simulink model "mcb_pmsm_foc_qep_f28379d_SIUnit"  (R2025b)
settings: Solver=FixedStepDiscrete  StartTime=0.0  StopTime=4  RelTol=1e-3  EnableMultiTasking=on
InitFcn:
  | mcb_pmsm_foc_qep_f28379d_SIUnit_data;
values from neighbouring files (symbols this model uses):
  A = [ -Rs/L,           0,                  0 ... (first row only)    [mcb_pmsm_fsfb_f28379d_param.m]    (also in v0_pmsm_fsfb_sim_for_flipsky_.m = [; v1_0_3_sim_param_fsfc.m = [)
  dataType = 'single'    [mcb_pmsm_foc_qep_f28379d_SIUnit_data.m]
  inverter = mcb.updateInverterParameters(pmsm,inverter,target)    [mcb_pmsm_foc_qep_f28379d_SIUnit_data.m]
  lambda_pm = pmsm.FluxPM    [mcb_pmsm_foc_qep_f28379d_SIUnit_data.m]
  PI_params = mcb.calcFOCGains(motor,Ts,Ts_speed,SpdLPFltCoeff=LPFltCoeff)    [mcb_pmsm_foc_qep_f28379d_SIUnit_data.m]
  pmsm = mcb.getPMSMParameters('Teknic2310P')    [mcb_pmsm_foc_qep_f28379d_SIUnit_data.m]
  T_pwm = 1/PWM_frequency    (= 5e-05)    [mcb_pmsm_foc_qep_f28379d_SIUnit_data.m]
  target = mcb.getProcessorParameters('F28379D',PWM_frequency)    [mcb_pmsm_foc_qep_f28379d_SIUnit_data.m]
  Ts = T_pwm    (= 5e-05)    [mcb_pmsm_foc_qep_f28379d_SIUnit_data.m]    (also in v0_pmsm_fsfb_sim_for_flipsky_.m = 0.0001; v1_0_3_sim_param_fsfc.m = 0.0001)
  Ts_inverter = T_pwm/2    (= 2.5e-05)    [mcb_pmsm_foc_qep_f28379d_SIUnit_data.m]
  Ts_motor = T_pwm/2    (= 2.5e-05)    [mcb_pmsm_foc_qep_f28379d_SIUnit_data.m]
  Ts_simulink = T_pwm/2    (= 2.5e-05)    [mcb_pmsm_foc_qep_f28379d_SIUnit_data.m]
  Ts_speed = 10*Ts    (= 0.0005)    [mcb_pmsm_foc_qep_f28379d_SIUnit_data.m]
undefined symbols (not defined in the file or in its folder): bit, DiscIntNeverNeededParam, Down, GPTRIP1SEL, GPTRIP2SEL, TZ1, TZ2, Up
libraries: mcbcontrolslib x8, c2802xlib x7, simulink x7, c280xlib x5, c2837xDlib x4, mcbeeMathTransformLib x3, slpidlib x3, mcbpositiondecoderlib x3, c2000lib x1, svdutilitieslib x1, autolibpmsmexterior x1
(part 2 of 2)

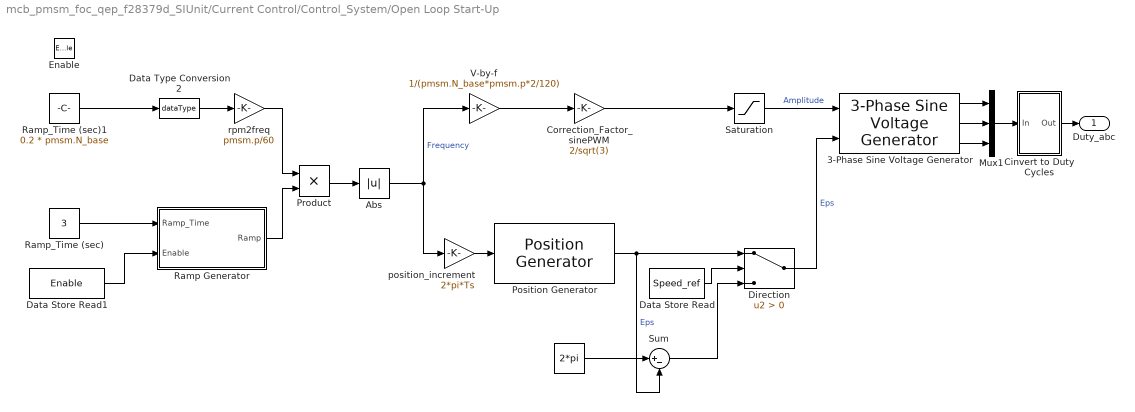
== system mcb_pmsm_foc_qep_f28379d_SIUnit/Current Control/Control_System/Open Loop Start-Up ==
  Enable : EnablePort  StatesWhenEnabling=reset
  " " : Constant  Value=2*pi  OutDataTypeStr=dataType  SampleTime=-1
  3-Phase Sine Voltage Generator : mcbcontrolslib/3-Phase Sine Voltage Generator  AngleInput=Radians  N_points=1024
  Abs : Abs  SaturateOnIntegerOverflow=off
  Cinvert to Duty Cycles : Subsystem
  Correction_Factor_sinePWM : Gain  Gain=2/sqrt(3)  RndMeth=Simplest  OutDataTypeStr=Inherit: Same as input
  Data Store Read : DataStoreRead  DataStoreName=Speed_ref  IndexOptions=Index vector (dialog)  Indices=1  OutputSizes=1
  Data Store Read1 : DataStoreRead  DataStoreName=Enable  IndexOptions=Index vector (dialog)  Indices=1  OutputSizes=1
  Data Type Conversion2 : DataTypeConversion  OutDataTypeStr=dataType  RndMeth=Simplest  SaturateOnIntegerOverflow=off
  Direction : Switch  Criteria=u2 > Threshold  OutDataTypeStr=dataType  RndMeth=Simplest  SaturateOnIntegerOverflow=off  InputSameDT=off
  Mux1 : Mux  Inputs=3
  Position Generator : mcbcontrolslib/Position Generator  AngleOutput=Radians  InitialThetaSource=Specify via dialog  ExternalReset=none  Offset=0
  Product : Product  RndMeth=Simplest  OutDataTypeStr=Inherit: Same as first input
  Ramp Generator : Subsystem
  Ramp_Time (sec) : Constant  Value=3  OutDataTypeStr=dataType  SampleTime=-1
  Ramp_Time (sec)1 : Constant  Value=0.2 * pmsm.N_base  OutDataTypeStr=dataType  SampleTime=-1
  Saturation : Saturate  UpperLimit=0.95  LowerLimit=0.15  RndMeth=Simplest
  Sum : Sum  Inputs=|+-  RndMeth=Simplest  OutDataTypeStr=Inherit: Same as first input
  V-by-f : Gain  Gain=1/(pmsm.N_base*pmsm.p*2/120)  RndMeth=Simplest  OutDataTypeStr=Inherit: Same as input
  position_increment : Gain  Gain=2*pi*Ts  RndMeth=Simplest  OutDataTypeStr=Inherit: Same as input
  rpm2freq : Gain  Gain=pmsm.p/60  RndMeth=Simplest  OutDataTypeStr=Inherit: Same as input
  Duty_abc : Outport  VectorParamsAs1DForOutWhenUnconnected=off
  wires:
  3-Phase Sine Voltage Generator/1 -> Mux1/1
  3-Phase Sine Voltage Generator/3 -> Mux1/3
  Direction/1 -> 3-Phase Sine Voltage Generator/2  "Eps"
  Saturation/1 -> 3-Phase Sine Voltage Generator/1  "Amplitude"
  Ramp Generator/1(Ramp) -> Product/2
  Ramp_Time (sec)/1 -> Ramp Generator/1(Ramp_Time)
  Position Generator/1 -> Sum/2, Direction/1  "Eps"
  " "/1 -> Sum/1
  Sum/1 -> Direction/3
  Abs/1 -> position_increment/1, V-by-f/1  "Frequency"
  position_increment/1 -> Position Generator/1
  V-by-f/1 -> Correction_Factor_sinePWM/1
  Product/1 -> Abs/1
  rpm2freq/1 -> Product/1
  Data Store Read1/1 -> Ramp Generator/2(Enable)
  Correction_Factor_sinePWM/1 -> Saturation/1
  3-Phase Sine Voltage Generator/2 -> Mux1/2
  Data Type Conversion2/1 -> rpm2freq/1
  Ramp_Time (sec)1/1 -> Data Type Conversion2/1
  Data Store Read/1 -> Direction/2
  Mux1/1 -> Cinvert to Duty Cycles/1(In)
  Cinvert to Duty Cycles/1(Out) -> Duty_abc/1

== system mcb_pmsm_foc_qep_f28379d_SIUnit/Current Control/HW_Inputs/Sensor Driver Blocks (codegen) ==
  Sim : Inport
  ADC_B_IN2 : c2802xlib/ADC  blkParamProc=C2000_Type4  ADCModule=B  samplingMode=Single sample mode  ADCResolution=12-bit (Single-ended input)  useSOC1=SOC0  useSOC2=SOC0_SOC1  SOCAcquisitionWindow=15  SOCTriggerSource=ePWM1_ADCSOCA  SOCInterruptTrigger=No ADCINT  Ts=-1  dType=uint16  postInterrupt=on  interruptSel=ADCINT1  ADCINTContinuous=on  endma=off  chdma=1  conv1=ADCINA0  conv2=ADCINA0 and ADCINB0  conv1_Type4=ADCIN2  conv2_Type4=ADCIN0 and ADCIN1
  ADC_C_IN2 : c2802xlib/ADC  blkParamProc=C2000_Type4  ADCModule=C  samplingMode=Single sample mode  ADCResolution=12-bit (Single-ended input)  useSOC1=SOC0  useSOC2=SOC0_SOC1  SOCAcquisitionWindow=15  SOCTriggerSource=ePWM1_ADCSOCA  SOCInterruptTrigger=No ADCINT  Ts=-1  dType=uint16  postInterrupt=off  interruptSel=ADCINT1  ADCINTContinuous=on  endma=off  chdma=1  conv1=ADCINA0  conv2=ADCINA0 and ADCINB0  conv1_Type4=ADCIN2  conv2_Type4=ADCIN0 and ADCIN1
  Mux1 : Mux
  Terminator : Terminator
  eQEP : c280xlib/eQEP  useModule=eQEP1  pcInputmode=Quadrature-count  externalClockrate=2x resolution: Count the rising/falling edge  swapPolarityselection=Clockwise  qdfOutputport=off  qapPolarityselection=on  qbpPolarityselection=on  qipPolarityselection=on  qspPolarityselection=off  igatePolarityselection=off  sampleTime=-1  pcOutputport=on  pcMaximumvalue=2^16-1  indexInitializationcheck=off  indexInitializationevent=Rising edge  strobeInitializationcheck=off  strobeInitializationevent=Rising edge  softwareInitializationcheck=off  softwareInitializationsource=Set to init value at start up  softwareInitializationmode=on  pcInitialvalue=2147483648  pcResetmode=Reset on the first index event  ieloutputport=on  indexEventlatch=Falling edge  seloutputport=off  strobeEventlatch=Rising edge  pcefOutputport=off  enableEqepcapture=off  qctmrOutputport=off  qcprdOutputport=off  captureTimerprescaler=128  upEventprescaler=128  overflowErrorflag=off  directionErrorflag=off  captureTimerposition=On position counter read  unitTimerperiod=100000000  captureTimerlatch=off  capturePeriodlatch=off  positionCounterlatch=off  soenPolarityselection=off  spselPolarityselection=Index pin is used for sync output  compareValuesource=Specify via dialog  shadowMode=Load on QPOSCNT=0  compareValue=4294967295  syncOutputwidth=1  polaritySyncoutput=Active high  watchdogEnable=off  watchdogTimer=65535  outport1Datatype=auto  outport2Datatype=auto  outport3Datatype=auto  outport4Datatype=auto  outport5Datatype=auto  outport6Datatype=auto  outport7Datatype=auto  outport8Datatype=auto  outport9Datatype=auto  outport10Datatype=auto  outport11Datatype=auto  outport12Datatype=auto  eqepinterrupt_pce=off  eqepinterrupt_qpe=off  eqepinterrupt_qdc=off  eqepinterrupt_wto=off  eqepinterrupt_pcu=off  eqepinterrupt_pco=off  eqepinterrupt_pcr=off  eqepinterrupt_pcm=off  eqepinterrupt_sel=off  eqepinterrupt_iel=off  eqepinterrupt_uto=off  pheOutputport=off  watchdogOutputport=off  outport13Datatype=auto  outport14Datatype=auto
  Out : Outport
  wires:
  ADC_C_IN2/1 -> Mux1/1
  Mux1/1 -> Out/1
  ADC_B_IN2/1 -> Mux1/2
  Sim/1 -> Terminator/1
  eQEP/1 -> Mux1/3
  eQEP/2 -> Mux1/4

== system mcb_pmsm_foc_qep_f28379d_SIUnit/Current Control/HW_Inputs/Sensor Driver Blocks (sim) ==
  Sim : Inport
  Out : Outport
  wires:
  Sim/1 -> Out/1

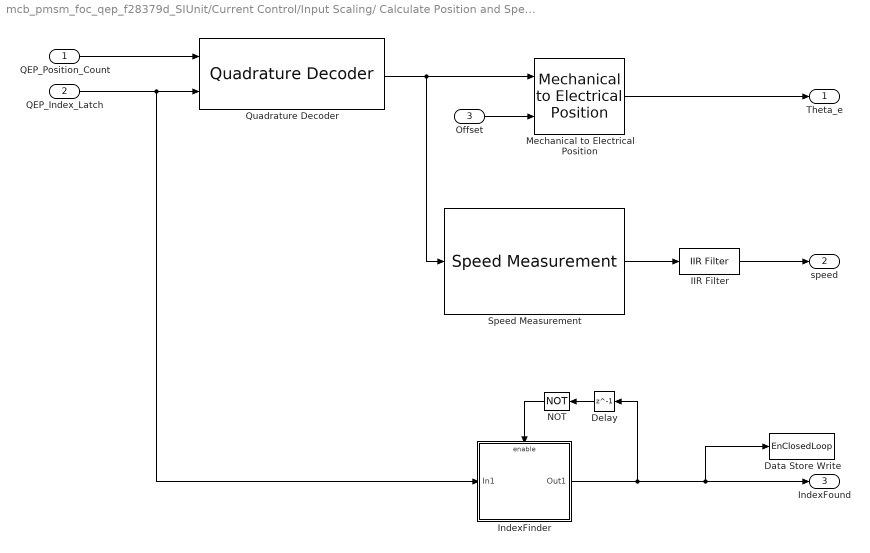
== system mcb_pmsm_foc_qep_f28379d_SIUnit/Current Control/Input Scaling/ Calculate Position and Speed ==
  QEP_Position_Count : Inport
  QEP_Index_Latch : Inport  Port=2
  Offset : Inport  Port=3
  Data Store Write : DataStoreWrite  DataStoreName=EnClosedLoop  IndexOptions=Index vector (dialog)  Indices=1  OutputSizes=1
  Delay : Delay  DelayLength=1
  IIR Filter : mcbcontrolslib/IIR Filter  VariantControl=Low Pass Filter  VariantSelect=Low-pass  FilterConstantInputType=Specify via dialog  Filter_constant=0.01  InitialOutput=Specify via dialog  InitialOutputValue=0  ExternalReset=none  advancedSettings=off  Ts=50e-6  cutOff_freq=32.1525
  IndexFinder : Subsystem
  Mechanical to Electrical Position : mcbpositiondecoderlib/Mechanical to Electrical Position  PolePairsInputType=Specify via dialog  NrPP=pmsm.p  selectedRange=Radians  MechOfstInputType=Input port  mechOffsetIn=0  maxAngleIn=2*pi  InputDataType=dataType  VariantSelect=floating-point
  NOT : Logic  Operator=NOT  AllPortsSameDT=off  OutDataTypeStr=boolean
  Quadrature Decoder : mcbpositiondecoderlib/Quadrature Decoder  ParameterInputType=off  CountsPerRevInverseDataType=single  EncoderSlitsPerRevolution=pmsm.QEPSlits  EncoderCountsPerSlit=4  CounterSize=16 bits  ExternalIndexCount=on  PositionUnit=Radians  PositionDataType=dataType
  Speed Measurement : mcbpositiondecoderlib/Speed Measurement  DiscreteStepInput=off  LastDiscreteStepInput=off  PositionUnit=Radians  PositionScalingDatatype=uint32  SpeedCalculationMode=Time interval for speed calculation  TempSpeedCalculationMode=Time interval for speed calculation  SampleTimeAsync=Ts  MaximumApplicationSpeed=6000  SpeedResolution=5e-6  DelayLength=20  MaximumMeasurableSpeed=29999  MeasurableSpeedResolution=1.397e-05  SpeedUnit=Radians/Sec  TempSpeedUnit=RPM  PerUnitSpeed=PU_System.N_base  SpeedDataType=dataType
  Theta_e : Outport  VectorParamsAs1DForOutWhenUnconnected=off
  speed : Outport  Port=2  VectorParamsAs1DForOutWhenUnconnected=off
  IndexFound : Outport  Port=3  InitialOutput=0  VectorParamsAs1DForOutWhenUnconnected=off
  wires:
  Speed Measurement/1 -> IIR Filter/1
  Mechanical to Electrical Position/1 -> Theta_e/1
  QEP_Position_Count/1 -> Quadrature Decoder/1
  Quadrature Decoder/1 -> Speed Measurement/1, Mechanical to Electrical Position/1
  Offset/1 -> Mechanical to Electrical Position/2
  IIR Filter/1 -> speed/1
  Delay/1 -> NOT/1
  NOT/1 -> IndexFinder/Enable
  IndexFinder/1(Out1) -> Data Store Write/1, IndexFound/1, Delay/1
  QEP_Index_Latch/1 -> IndexFinder/1(In1), Quadrature Decoder/2

== system mcb_pmsm_foc_qep_f28379d_SIUnit/Current Control/Input Scaling/Calculate Phase Currents ==
  Ia_ADC : Inport
  Ib_ADC : Inport  Port=2
  Add : Sum  Inputs=-+
  Data Store Read1 : DataStoreRead  DataStoreName=IaOffset  IndexOptions=Index vector (dialog)  Indices=1  OutputSizes=1
  Data Store Read2 : DataStoreRead  DataStoreName=IbOffset  IndexOptions=Index vector (dialog)  Indices=1  OutputSizes=1
  Data Type Conversion : DataTypeConversion  OutDataTypeStr=int32  ConvertRealWorld=Stored Integer (SI)  RndMeth=Simplest  SaturateOnIntegerOverflow=off
  Get ADC Voltage : Gain  Gain=target.ADC_Vref /target.ADC_MaxCount  OutDataTypeStr=dataType  RndMeth=Simplest
  Get Currents : Gain  Gain=inverter.invertingAmp/inverter.ISenseVoltPerAmp  RndMeth=Simplest  OutDataTypeStr=Inherit: Same as input
  Mux : Mux  Inputs=2
  Mux1 : Mux  Inputs=2
  Iab_meas : Outport  VectorParamsAs1DForOutWhenUnconnected=off
  wires:
  Data Type Conversion/1 -> Add/2
  Ia_ADC/1 -> Mux/1
  Ib_ADC/1 -> Mux/2
  Mux/1 -> Data Type Conversion/1
  Data Store Read1/1 -> Mux1/1
  Data Store Read2/1 -> Mux1/2
  Mux1/1 -> Add/1
  Get Currents/1 -> Iab_meas/1
  Get ADC Voltage/1 -> Get Currents/1
  Add/1 -> Get ADC Voltage/1

== system mcb_pmsm_foc_qep_f28379d_SIUnit/Current Control/SCI (Code Generation)/Data_Conditioning_Tx ==
  In1 : Inport
  Data_Type_Fixed_Point : Subsystem  VariantControl=~isequal(dataType,'single')
  Data_Type_Float : Subsystem  VariantControl=isequal(dataType, 'single')
  Data_Log : Outport

== system mcb_pmsm_foc_qep_f28379d_SIUnit/Current Control/SCI (Code Generation)/Data_Logging ==
  note: Fast Serial Data Monitoring (32-bit)
  Data_Log : Inport
  Counter Limited : simulink/Sources/Counter Limited  uplimit=600-1  tsamp=-1
  Data : Subsystem  TreatAsAtomicUnit=on
  End : Subsystem  TreatAsAtomicUnit=on
  If : If  IfExpression=u1 == 0  ElseIfExpressions=u1 == 599
  Merge : Merge  Inputs=3
  Merge1 : Merge  Inputs=3
  Mux : Mux  Inputs=2
  Start : Subsystem  TreatAsAtomicUnit=on
  Width : Width  OutDataTypeMode=All ports same datatype  DataType=uint16
  SCI_Tx : Outport
  wires:
  If/3 -> Data/Action
  Data/1(Data_out) -> Merge/3
  Width/1 -> Data/2(Data_width), Start/2(Data_width), End/2(Data_width)
  Merge/1 -> Mux/1  "SCI_Tx_Data"
  Counter Limited/1 -> If/1
  Start/2(Iteration) -> Merge1/1
  Start/1(Data_out) -> Merge/1
  If/2 -> End/Action
  Merge1/1 -> Mux/2  "SCI_Tx_Iteration"
  If/1 -> Start/Action
  End/1(Data_out) -> Merge/2
  End/2(Iteration) -> Merge1/2
  Data/2(Iteration) -> Merge1/3
  Mux/1 -> SCI_Tx/1
  Data_Log/1 -> Width/1, Start/1(Data), End/1(Data), Data/1(Data)

== system mcb_pmsm_foc_qep_f28379d_SIUnit/Current Control/SCI (Code Generation)/While Iterator Subsystem ==
  Data : Inport
  Iteration : Inport  Port=2
  Add : Sum  Inputs=+-  OutDataTypeStr=Inherit: Same as first input
  Index Vector : MultiPortSwitch  Inputs=1  SaturateOnIntegerOverflow=off  InputSameDT=off
  SCI Transmit : c280xlib/SCI Transmit  sciModule=A  dataHead=''  dataTail=''  frameSize=1  blockingMode=on  outputStatus=off
  While Iterator : WhileIterator  MaxIters=-1  WhileBlockType=do-while  ShowIterationPort=on  OutputDataType=int16
  wires:
  While Iterator/1 -> Add/2, Index Vector/1
  Data/1 -> Index Vector/2
  Index Vector/1 -> SCI Transmit/1
  Add/1 -> While Iterator/1
  Iteration/1 -> Add/1

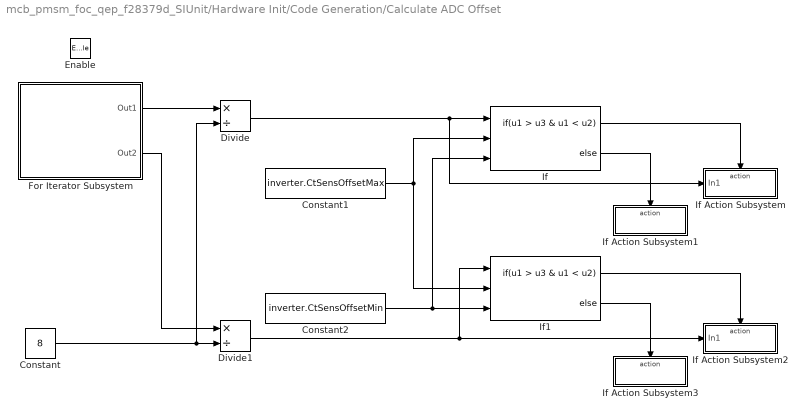
== system mcb_pmsm_foc_qep_f28379d_SIUnit/Hardware Init/Code Generation/Calculate ADC Offset  ==
  Enable : EnablePort
  Constant : Constant  Value=8
  Constant1 : Constant  Value=inverter.CtSensOffsetMax  OutDataTypeStr=Inherit: Inherit via back propagation
  Constant2 : Constant  Value=inverter.CtSensOffsetMin  OutDataTypeStr=Inherit: Inherit via back propagation
  Divide : Product  Inputs=*/  OutDataTypeStr=uint16
  Divide1 : Product  Inputs=*/  OutDataTypeStr=uint16
  For Iterator Subsystem : Subsystem  TreatAsAtomicUnit=on
  If : If  NumInputs=3  IfExpression=u1 > u3 & u1 < u2
  If Action Subsystem : Subsystem  TreatAsAtomicUnit=on
  If Action Subsystem1 : Subsystem  TreatAsAtomicUnit=on
  If Action Subsystem2 : Subsystem  TreatAsAtomicUnit=on
  If Action Subsystem3 : Subsystem  TreatAsAtomicUnit=on
  If1 : If  NumInputs=3  IfExpression=u1 > u3 & u1 < u2
  wires:
  For Iterator Subsystem/1(Out1) -> Divide/1
  If1/2 -> If Action Subsystem3/Action
  If1/1 -> If Action Subsystem2/Action
  Constant1/1 -> If/2, If1/2
  If/2 -> If Action Subsystem1/Action
  For Iterator Subsystem/2(Out2) -> Divide1/1
  If/1 -> If Action Subsystem/Action
  Constant2/1 -> If/3, If1/3
  Divide1/1 -> If Action Subsystem2/1(In1), If1/1
  Constant/1 -> Divide1/2, Divide/2
  Divide/1 -> If Action Subsystem/1(In1), If/1

== system mcb_pmsm_foc_qep_f28379d_SIUnit/Hardware Init/Code Generation/DRV Enable ==
  note: Enable Inverter
  In : Inport
  ADC Gain Setting : Subsystem
  Constant : Constant  Value=inverter.EnableLogic
  DRV830x Enable : Constant  OutDataTypeStr=uint16  SampleTime=-1
  Digital Output : c2837xDlib/Digital Output  Priority=10  GPIO_Number=GPIO120~GPIO127  GPIO_Bit0=off  GPIO_BIT0_Toggle=off  GPIO_Bit1=off  GPIO_BIT1_Toggle=off  GPIO_Bit2=off  GPIO_BIT2_Toggle=off  GPIO_Bit3=off  GPIO_BIT3_Toggle=off  GPIO_Bit4=on  GPIO_BIT4_Toggle=off  GPIO_Bit5=off  GPIO_BIT5_Toggle=off  GPIO_Bit6=off  GPIO_BIT6_Toggle=off  GPIO_Bit7=off  GPIO_BIT7_Toggle=off
  Digital Output1 : c2837xDlib/Digital Output  Priority=10  GPIO_Number=GPIO16~GPIO23  GPIO_Bit0=off  GPIO_BIT0_Toggle=off  GPIO_Bit1=off  GPIO_BIT1_Toggle=off  GPIO_Bit2=off  GPIO_BIT2_Toggle=off  GPIO_Bit3=off  GPIO_BIT3_Toggle=off  GPIO_Bit4=off  GPIO_BIT4_Toggle=off  GPIO_Bit5=off  GPIO_BIT5_Toggle=off  GPIO_Bit6=on  GPIO_BIT6_Toggle=off  GPIO_Bit7=off  GPIO_BIT7_Toggle=off
  NOT : Logic  Operator=NOT  IconShape=distinctive  AllPortsSameDT=off  OutDataTypeStr=boolean
  RunTimeMeasurement : Constant  OutDataTypeStr=uint16  SampleTime=-1
  Switch : Switch  Criteria=u2 > Threshold  SaturateOnIntegerOverflow=off  InputSameDT=off
  wires:
  RunTimeMeasurement/1 -> Digital Output1/1
  Switch/1 -> Digital Output/1
  DRV830x Enable/1 -> NOT/1, Switch/1
  NOT/1 -> Switch/3
  Constant/1 -> ADC Gain Setting/Enable, Switch/2
  In/1 -> ADC Gain Setting/1(In)

== system mcb_pmsm_foc_qep_f28379d_SIUnit/Hardware Init/Code Generation/Default ADC Offset ==
  Enable : EnablePort
  Constant : Constant  Value=inverter.CtSensAOffset  OutDataTypeStr=Inherit: Inherit via back propagation
  Constant1 : Constant  Value=inverter.CtSensBOffset  OutDataTypeStr=Inherit: Inherit via back propagation
  Data Store Write1 : DataStoreWrite  DataStoreName=IaOffset  IndexOptions=Index vector (dialog)  Indices=1  OutputSizes=1
  Data Store Write2 : DataStoreWrite  DataStoreName=IbOffset  IndexOptions=Index vector (dialog)  Indices=1  OutputSizes=1
  wires:
  Constant/1 -> Data Store Write1/1
  Constant1/1 -> Data Store Write2/1

== system mcb_pmsm_foc_qep_f28379d_SIUnit/Inverter and Motor - Plant Model/Simulation/Inverter ==
  Duty_abc : Inport
  Average_Value_Inverter : Subsystem
  Constant2 : Constant  Value=inverter.V_dc  OutDataTypeStr=single  SampleTime=-1
  Data Type Conversion1 : DataTypeConversion  OutDataTypeStr=single  RndMeth=Simplest  SaturateOnIntegerOverflow=off
  Demux : Demux  Outputs=3
  Inverter_delay : DiscreteTransferFcn  Numerator=[1-exp(-Ts_inverter/(T_pwm/2))]  Denominator=[1 -exp(-Ts_inverter/(T_pwm/2))]  RndMeth=Simplest
  Mux : Mux  Inputs=3
  Rate Transition3 : RateTransition  Integrity=off  OutPortSampleTime=Ts_inverter
  Vabc : Outport  VectorParamsAs1DForOutWhenUnconnected=off
  wires:
  Average_Value_Inverter/2(Vb) -> Mux/2
  Mux/1 -> Inverter_delay/1
  Constant2/1 -> Average_Value_Inverter/4(Vdc)
  Average_Value_Inverter/3(Vc) -> Mux/3
  Average_Value_Inverter/1(Va) -> Mux/1
  Demux/1 -> Average_Value_Inverter/1(Vao)
  Demux/3 -> Average_Value_Inverter/3(Vco)
  Demux/2 -> Average_Value_Inverter/2(Vbo)
  Data Type Conversion1/1 -> Rate Transition3/1
  Rate Transition3/1 -> Demux/1
  Inverter_delay/1 -> Vabc/1
  Duty_abc/1 -> Data Type Conversion1/1

== system mcb_pmsm_foc_qep_f28379d_SIUnit/Inverter and Motor - Plant Model/Simulation/Load_Profile (Torque) ==
  Data Type Conversion : DataTypeConversion  OutDataTypeStr=single  SaturateOnIntegerOverflow=off  RndMeth=Floor
  IIR Filter : mcbcontrolslib/IIR Filter  VariantControl=Low Pass Filter  VariantSelect=Low-pass  FilterConstantInputType=Specify via dialog  Filter_constant=0.01  InitialOutput=Specify via dialog  InitialOutputValue=0  ExternalReset=none  advancedSettings=off  Ts=50e-6  cutOff_freq=32.1525
  T_load : Step  Time=2  Before=0.05*pmsm.T_rated  After=0.5*pmsm.T_rated  SampleTime=Ts_simulink
  Load_Trq : Outport  VectorParamsAs1DForOutWhenUnconnected=off
  wires:
  Data Type Conversion/1 -> IIR Filter/1
  T_load/1 -> Data Type Conversion/1
  IIR Filter/1 -> Load_Trq/1

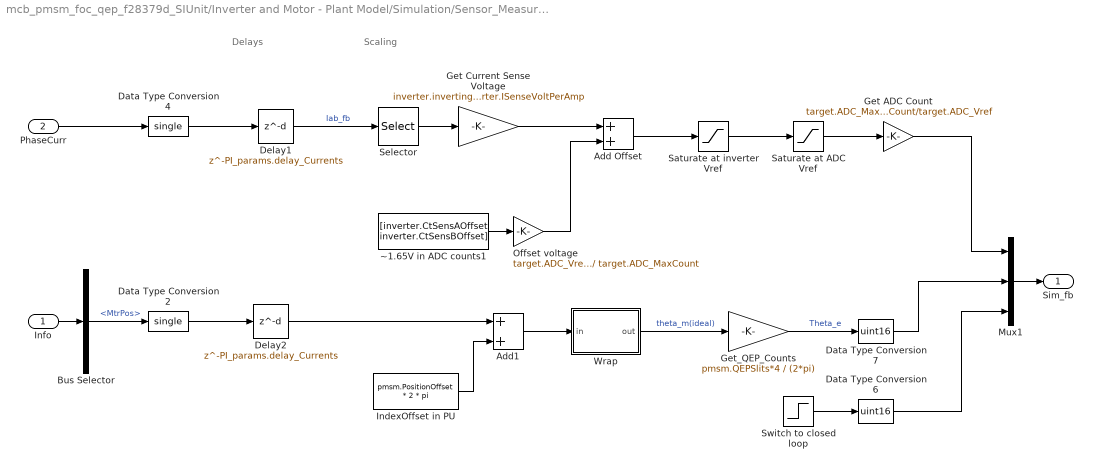
== system mcb_pmsm_foc_qep_f28379d_SIUnit/Inverter and Motor - Plant Model/Simulation/Sensor_Measurements ==
  note: Scaling
  note: Delays
  Info : Inport
  PhaseCurr : Inport  Port=2
  Add Offset : Sum  RndMeth=Simplest
  Add1 : Sum  RndMeth=Simplest
  Bus Selector : BusSelector  OutputSignals=MtrPos
  Data Type Conversion2 : DataTypeConversion  OutDataTypeStr=single  RndMeth=Simplest  SaturateOnIntegerOverflow=off
  Data Type Conversion4 : DataTypeConversion  OutDataTypeStr=single  RndMeth=Simplest  SaturateOnIntegerOverflow=off
  Data Type Conversion6 : DataTypeConversion  OutDataTypeStr=uint16  RndMeth=Simplest  SaturateOnIntegerOverflow=off
  Data Type Conversion7 : DataTypeConversion  OutDataTypeStr=uint16  RndMeth=Simplest  SaturateOnIntegerOverflow=off
  Delay1 : Delay  DelayLength=PI_params.delay_Currents
  Delay2 : Delay  DelayLength=PI_params.delay_Currents
  Get ADC Count : Gain  Gain=target.ADC_MaxCount/target.ADC_Vref  OutMin=0  OutMax=target.ADC_MaxCount  OutDataTypeStr=uint16  RndMeth=Simplest
  Get Current Sense Voltage : Gain  Gain=inverter.invertingAmp * inverter.ISenseVoltPerAmp  RndMeth=Simplest  OutDataTypeStr=Inherit: Same as input
  Get_QEP_Counts : Gain  Gain=pmsm.QEPSlits*4 / (2*pi)  OutDataTypeStr=uint16  RndMeth=Simplest
  IndexOffset in PU : Constant  Value=pmsm.PositionOffset * 2 * pi  OutDataTypeStr=single  SampleTime=-1
  Mux1 : Mux  Inputs=3
  Offset voltage : Gain  Gain=target.ADC_Vref / target.ADC_MaxCount  RndMeth=Simplest
  Saturate at ADC Vref : Saturate  UpperLimit=target.ADC_Vref  LowerLimit=0
  Saturate at inverter Vref : Saturate  UpperLimit=inverter.ISenseVref  LowerLimit=0
  Selector : Selector  InputPortWidth=3  IndexOptions=Index vector (dialog)  Indices=[1 2]  OutputSizes=1
  Switch to closed loop : Step  Time=0.1  SampleTime=Ts_motor
  Wrap : Subsystem
  ~1.65V in ADC counts1 : Constant  Value=[inverter.CtSensAOffset inverter.CtSensBOffset]  OutDataTypeStr=uint16  SampleTime=-1
  Sim_fb : Outport  VectorParamsAs1DForOutWhenUnconnected=off
  wires:
  Delay1/1 -> Selector/1  "Iab_fb"
  Data Type Conversion4/1 -> Delay1/1
  PhaseCurr/1 -> Data Type Conversion4/1
  Info/1 -> Bus Selector/1
  Bus Selector/1 -> Data Type Conversion2/1  "<MtrPos>"
  Data Type Conversion2/1 -> Delay2/1
  Mux1/1 -> Sim_fb/1
  Delay2/1 -> Add1/1
  IndexOffset in PU/1 -> Add1/2
  Add1/1 -> Wrap/1(in)
  Get_QEP_Counts/1 -> Data Type Conversion7/1  "Theta_e"
  Wrap/1(out) -> Get_QEP_Counts/1  "theta_m(ideal)"
  Switch to closed loop/1 -> Data Type Conversion6/1
  ~1.65V in ADC counts1/1 -> Offset voltage/1
  Get Current Sense Voltage/1 -> Add Offset/1
  Saturate at ADC Vref/1 -> Get ADC Count/1
  Add Offset/1 -> Saturate at inverter Vref/1
  Saturate at inverter Vref/1 -> Saturate at ADC Vref/1
  Selector/1 -> Get Current Sense Voltage/1
  Offset voltage/1 -> Add Offset/2
  Data Type Conversion6/1 -> Mux1/3
  Data Type Conversion7/1 -> Mux1/2
  Get ADC Count/1 -> Mux1/1

== system mcb_pmsm_foc_qep_f28379d_SIUnit/Serial Receive/Data_Conditioning_Rx/Data_Type_Fixed_Point ==
  In1 : Inport
  Data Type Conversion1 : DataTypeConversion  OutDataTypeStr=dataType  RndMeth=Simplest  SaturateOnIntegerOverflow=off
  Data Type Conversion2 : DataTypeConversion  OutDataTypeStr=fixdt(1,32,28)  ConvertRealWorld=Stored Integer (SI)  RndMeth=Simplest  SaturateOnIntegerOverflow=off
  Data Type Conversion3 : DataTypeConversion  OutDataTypeStr=uint16  RndMeth=Simplest  SaturateOnIntegerOverflow=off
  Demux : Demux  Outputs=2
  Desired Speed : Outport
  Out2 : Outport  Port=2
  wires:
  In1/1 -> Demux/1
  Data Type Conversion1/1 -> Desired Speed/1
  Data Type Conversion2/1 -> Data Type Conversion1/1
  Demux/1 -> Data Type Conversion2/1
  Demux/2 -> Data Type Conversion3/1
  Data Type Conversion3/1 -> Out2/1

== system mcb_pmsm_foc_qep_f28379d_SIUnit/Serial Receive/Data_Conditioning_Rx/Data_Type_Float ==
  In1 : Inport
  Data Type Conversion2 : DataTypeConversion  OutDataTypeStr=uint16  RndMeth=Simplest  SaturateOnIntegerOverflow=off
  Demux : Demux  Outputs=2
  Desired Speed : Outport
  Out2 : Outport  Port=2
  wires:
  In1/1 -> Demux/1
  Demux/1 -> Desired Speed/1
  Data Type Conversion2/1 -> Out2/1
  Demux/2 -> Data Type Conversion2/1

== system mcb_pmsm_foc_qep_f28379d_SIUnit/Serial Receive/Simulation/Data_Conditioning_Tx ==
  In1 : Inport
  In2 : Inport  Port=2
  Data_Type_Fixed_Point : Subsystem  VariantControl=~isequal(dataType, 'single')
  Data_Type_Float : Subsystem  VariantControl=isequal(dataType, 'single')
  Data : Outport

== system mcb_pmsm_foc_qep_f28379d_SIUnit/Serial Receive/Simulation/Parse ==
  Enable_PWM : Inport
  Debug_signals : Inport  Port=2
  Bitwise Operator : simulink/Logic and Bit Operations/Bitwise Operator  logicop=AND  UseBitMask=on  BitMask=hex2dec('0001')  BitMaskRealWorld=Stored Integer
  Bitwise Operator1 : simulink/Logic and Bit Operations/Bitwise Operator  logicop=AND  UseBitMask=on  BitMask=hex2dec('00F0')  BitMaskRealWorld=Stored Integer
  Shift Arithmetic1 : ArithShift  BitShiftNumber=-4
  Sum : Sum
  Data : Outport
  wires:
  Bitwise Operator/1 -> Sum/1
  Debug_signals/1 -> Shift Arithmetic1/1
  Sum/1 -> Data/1
  Shift Arithmetic1/1 -> Bitwise Operator1/1
  Enable_PWM/1 -> Bitwise Operator/1
  Bitwise Operator1/1 -> Sum/2

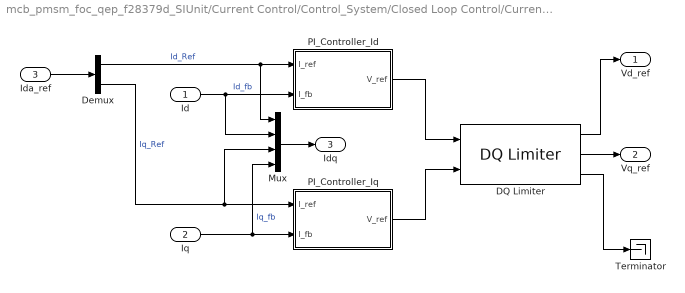
== system mcb_pmsm_foc_qep_f28379d_SIUnit/Current Control/Control_System/Closed Loop Control/Current_Controllers ==
  Id : Inport
  Iq : Inport  Port=2
  Ida_ref : Inport  Port=3
  DQ Limiter : mcbcontrolslib/DQ Limiter  satMethodInputType=Specify via dialog  satMethodSelected=D-Q equivalence  satLimitInputType=Specify via dialog  Vmax=inverter.V_dc/sqrt(3) *0.95
  Demux : Demux  Outputs=2
  Mux : Mux
  PI_Controller_Id : Subsystem
  PI_Controller_Iq : Subsystem
  Terminator : Terminator
  Vd_ref : Outport  VectorParamsAs1DForOutWhenUnconnected=off
  Vq_ref : Outport  Port=2  VectorParamsAs1DForOutWhenUnconnected=off
  Idq : Outport  Port=3  VectorParamsAs1DForOutWhenUnconnected=off
  wires:
  Iq/1 -> Mux/4, PI_Controller_Iq/2(I_fb)  "Iq_fb"
  Id/1 -> Mux/2, PI_Controller_Id/2(I_fb)  "Id_fb"
  Demux/1 -> Mux/1, PI_Controller_Id/1(I_ref)  "Id_Ref"
  Demux/2 -> Mux/3, PI_Controller_Iq/1(I_ref)  "Iq_Ref"
  Ida_ref/1 -> Demux/1
  Mux/1 -> Idq/1
  PI_Controller_Id/1(V_ref) -> DQ Limiter/1
  PI_Controller_Iq/1(V_ref) -> DQ Limiter/2
  DQ Limiter/2 -> Vq_ref/1
  DQ Limiter/1 -> Vd_ref/1
  DQ Limiter/3 -> Terminator/1

== system mcb_pmsm_foc_qep_f28379d_SIUnit/Current Control/Control_System/Closed Loop Control/SVPWM ==
  Va : Inport
  Vb : Inport  Port=2
  Constant : Constant  Value=0.5  OutDataTypeStr=dataType  SampleTime=-1
  Gain : Gain  Gain=1/ (2 * inverter.V_dc / sqrt(3))  RndMeth=Simplest  OutDataTypeStr=Inherit: Same as input
  Mux1 : Mux  Inputs=3
  Space Vector Generator : mcbcontrolslib/PWM Reference Generator  inSignal=Valphabeta  modType=SVM: space vector modulation
  Sum : Sum  Inputs=|++
  Duty_abc : Outport
  wires:
  Va/1 -> Space Vector Generator/1
  Space Vector Generator/2 -> Mux1/2
  Space Vector Generator/3 -> Mux1/3
  Space Vector Generator/1 -> Mux1/1
  Vb/1 -> Space Vector Generator/2
  Gain/1 -> Sum/1
  Constant/1 -> Sum/2
  Sum/1 -> Duty_abc/1
  Mux1/1 -> Gain/1

== system mcb_pmsm_foc_qep_f28379d_SIUnit/Current Control/Control_System/Open Loop Start-Up/Cinvert to Duty Cycles ==
  In : Inport
  Constant : Constant  Value=0.5  OutDataTypeStr=dataType  SampleTime=-1
  Normalize : Gain  Gain=1/2
  Sum : Sum  Inputs=|++
  Out : Outport
  wires:
  In/1 -> Normalize/1
  Normalize/1 -> Sum/1
  Constant/1 -> Sum/2
  Sum/1 -> Out/1

== system mcb_pmsm_foc_qep_f28379d_SIUnit/Current Control/Control_System/Open Loop Start-Up/Ramp Generator ==
  Ramp_Time : Inport
  Enable : Inport  Port=2
  Divide : Product  Inputs=*/  RndMeth=Simplest  OutDataTypeStr=Inherit: Same as first input
  NOT : Logic  Operator=NOT  IconShape=distinctive  AllPortsSameDT=off  OutDataTypeStr=boolean
  One : Constant  OutDataTypeStr=dataType  SampleTime=-1
  Ramp Generator : DiscreteIntegrator  IntegratorMethod=Accumulation: Forward Euler  gainval=1  ExternalReset=sampled level  SampleTime=-1  OutDataTypeStr=dataType  RndMeth=Simplest  LimitOutput=on  UpperSaturationLimit=1  LowerSaturationLimit=0  ICPrevOutput=DiscIntNeverNeededParam  ICPrevScaledInput=DiscIntNeverNeededParam
  Sample_Time : Gain  Gain=Ts  RndMeth=Simplest  OutDataTypeStr=Inherit: Same as input
  Ramp : Outport
  wires:
  Divide/1 -> Sample_Time/1
  Ramp Generator/1 -> Ramp/1  "Eps"
  Sample_Time/1 -> Ramp Generator/1
  One/1 -> Divide/1
  Ramp_Time/1 -> Divide/2
  Enable/1 -> NOT/1
  NOT/1 -> Ramp Generator/2

== system mcb_pmsm_foc_qep_f28379d_SIUnit/Current Control/Input Scaling/ Calculate Position and Speed/IndexFinder ==
  In1 : Inport
  Enable : EnablePort
  AND : Logic  AllPortsSameDT=off  OutDataTypeStr=boolean
  Compare To Constant : simulink/Logic and Bit Operations/Compare To Constant  relop===  const=0  OutDataTypeStr=boolean
  Compare To Constant1 : simulink/Logic and Bit Operations/Compare To Constant  relop=>  const=0  OutDataTypeStr=boolean
  Delay3 : Delay  DelayLength=1
  Out1 : Outport
  wires:
  In1/1 -> Delay3/1, Compare To Constant1/1
  Compare To Constant1/1 -> AND/2
  Compare To Constant/1 -> AND/1
  Delay3/1 -> Compare To Constant/1
  AND/1 -> Out1/1

== system mcb_pmsm_foc_qep_f28379d_SIUnit/Current Control/SCI (Code Generation)/Data_Conditioning_Tx/Data_Type_Fixed_Point ==
  In1 : Inport
  Data Type Conversion : DataTypeConversion  OutDataTypeStr=fixdt(1,32,28)  RndMeth=Simplest  SaturateOnIntegerOverflow=off
  Data Type Conversion3 : DataTypeConversion  OutDataTypeStr=uint32  ConvertRealWorld=Stored Integer (SI)  RndMeth=Simplest  SaturateOnIntegerOverflow=off
  Data_Log : Outport
  wires:
  In1/1 -> Data Type Conversion/1
  Data Type Conversion3/1 -> Data_Log/1
  Data Type Conversion/1 -> Data Type Conversion3/1

== system mcb_pmsm_foc_qep_f28379d_SIUnit/Current Control/SCI (Code Generation)/Data_Conditioning_Tx/Data_Type_Float ==
  In1 : Inport
  Byte Pack : svdutilitieslib/Byte Pack  maskPackedDataType=uint32  datatypes={'single'}  byteAlign=4  blockPlatform=tic2000
  Data_Log : Outport
  wires:
  Byte Pack/1 -> Data_Log/1
  In1/1 -> Byte Pack/1

== system mcb_pmsm_foc_qep_f28379d_SIUnit/Current Control/SCI (Code Generation)/Data_Logging/Data ==
  Data : Inport
  Data_width : Inport  Port=2
  Action Port : ActionPort  ActionPortLabel=else
  Dummy : Constant  Value=hex2dec('0000')  OutDataTypeStr=uint32
  Mux : Mux  Inputs=2
  Data_out : Outport  VectorParamsAs1DForOutWhenUnconnected=off
  Iteration : Outport  Port=2  VectorParamsAs1DForOutWhenUnconnected=off
  wires:
  Data_width/1 -> Iteration/1
  Data/1 -> Mux/1
  Dummy/1 -> Mux/2
  Mux/1 -> Data_out/1

== system mcb_pmsm_foc_qep_f28379d_SIUnit/Current Control/SCI (Code Generation)/Data_Logging/End ==
  Data : Inport
  Data_width : Inport  Port=2
  Action Port : ActionPort  ActionPortLabel=elseif(u1 == 599)
  Bias : Bias  Bias=1  SaturateOnIntegerOverflow=off
  End : Constant  Value=hex2dec('45454545')  OutDataTypeStr=uint32
  Mux : Mux  Inputs=2
  Data_out : Outport  VectorParamsAs1DForOutWhenUnconnected=off
  Iteration : Outport  Port=2  VectorParamsAs1DForOutWhenUnconnected=off
  wires:
  Data/1 -> Mux/1
  Data_width/1 -> Bias/1
  Bias/1 -> Iteration/1
  End/1 -> Mux/2
  Mux/1 -> Data_out/1

== system mcb_pmsm_foc_qep_f28379d_SIUnit/Current Control/SCI (Code Generation)/Data_Logging/Start ==
  Data : Inport
  Data_width : Inport  Port=2
  Action Port : ActionPort  ActionPortLabel=if(u1 == 0)
  Bias : Bias  Bias=1  SaturateOnIntegerOverflow=off
  Mux : Mux  Inputs=2
  Start : Constant  Value=hex2dec('53535353')  OutDataTypeStr=uint32
  Data_out : Outport  VectorParamsAs1DForOutWhenUnconnected=off
  Iteration : Outport  Port=2  VectorParamsAs1DForOutWhenUnconnected=off
  wires:
  Data/1 -> Mux/2
  Data_width/1 -> Bias/1
  Bias/1 -> Iteration/1
  Start/1 -> Mux/1
  Mux/1 -> Data_out/1

== system mcb_pmsm_foc_qep_f28379d_SIUnit/Hardware Init/Code Generation/Calculate ADC Offset /For Iterator Subsystem ==
  ADC_A_IN0 : c2802xlib/ADC  Priority=20  blkParamProc=C2000_Type4  ADCModule=C  samplingMode=Single sample mode  ADCResolution=12-bit (Single-ended input)  ADC29xResolution=12-bit  ADCMode=Single-ended input  useSOC1=SOC2  useSOC2=SOC0_SOC1  SOCAcquisitionWindow=15  SOCTriggerSource=Software  SOCInterruptTrigger=No ADCINT  Ts=-1  dType=uint16  postInterrupt=off  interruptSel=ADCINT1  ADCINTContinuous=on  endma=off  chdma=1  conv1=ADCINA0  conv2=ADCINA0 and ADCINB0  conv1_Type4=ADCIN2  conv2_Type4=ADCIN0 and ADCIN1
  ADC_B_IN0 : c2802xlib/ADC  Priority=20  blkParamProc=C2000_Type4  ADCModule=B  samplingMode=Single sample mode  ADCResolution=12-bit (Single-ended input)  ADC29xResolution=12-bit  ADCMode=Single-ended input  useSOC1=SOC2  useSOC2=SOC0_SOC1  SOCAcquisitionWindow=15  SOCTriggerSource=Software  SOCInterruptTrigger=No ADCINT  Ts=-1  dType=uint16  postInterrupt=off  interruptSel=ADCINT1  ADCINTContinuous=on  endma=off  chdma=1  conv1=ADCINA0  conv2=ADCINA0 and ADCINB0  conv1_Type4=ADCIN2  conv2_Type4=ADCIN0 and ADCIN1
  For Iterator : ForIterator  IterationLimit=16  IterationVariableDataType=uint16
  If : If  IfExpression=u1 > 8  ShowElse=off
  If Action Subsystem : Subsystem  TreatAsAtomicUnit=on
  Out1 : Outport
  Out2 : Outport  Port=2
  wires:
  For Iterator/1 -> If/1
  ADC_A_IN0/1 -> If Action Subsystem/1(In1)
  ADC_B_IN0/1 -> If Action Subsystem/2(In2)
  If Action Subsystem/1(Out1) -> Out1/1
  If Action Subsystem/2(Out2) -> Out2/1
  If/1 -> If Action Subsystem/Action

== system mcb_pmsm_foc_qep_f28379d_SIUnit/Hardware Init/Code Generation/Calculate ADC Offset /If Action Subsystem ==
  In1 : Inport
  Action Port : ActionPort  ActionPortLabel=if(u1 > 2000 & u1 < 3000)
  Data Store Write1 : DataStoreWrite  DataStoreName=IaOffset  IndexOptions=Index vector (dialog)  Indices=1  OutputSizes=1
  wires:
  In1/1 -> Data Store Write1/1

== system mcb_pmsm_foc_qep_f28379d_SIUnit/Hardware Init/Code Generation/Calculate ADC Offset /If Action Subsystem1 ==
  Action Port : ActionPort  ActionPortLabel=else
  Constant : Constant  Value=inverter.CtSensAOffset  OutDataTypeStr=Inherit: Inherit via back propagation
  Data Store Write1 : DataStoreWrite  DataStoreName=IaOffset  IndexOptions=Index vector (dialog)  Indices=1  OutputSizes=1
  wires:
  Constant/1 -> Data Store Write1/1

== system mcb_pmsm_foc_qep_f28379d_SIUnit/Hardware Init/Code Generation/Calculate ADC Offset /If Action Subsystem2 ==
  In1 : Inport
  Action Port : ActionPort  ActionPortLabel=if(u1 > 2000 & u1 < 3000)
  Data Store Write2 : DataStoreWrite  DataStoreName=IbOffset  IndexOptions=Index vector (dialog)  Indices=1  OutputSizes=1
  wires:
  In1/1 -> Data Store Write2/1

== system mcb_pmsm_foc_qep_f28379d_SIUnit/Hardware Init/Code Generation/Calculate ADC Offset /If Action Subsystem3 ==
  Action Port : ActionPort  ActionPortLabel=else
  Constant1 : Constant  Value=inverter.CtSensBOffset  OutDataTypeStr=Inherit: Inherit via back propagation
  Data Store Write2 : DataStoreWrite  DataStoreName=IbOffset  IndexOptions=Index vector (dialog)  Indices=1  OutputSizes=1
  wires:
  Constant1/1 -> Data Store Write2/1

== system mcb_pmsm_foc_qep_f28379d_SIUnit/Hardware Init/Code Generation/DRV Enable/ADC Gain Setting ==
  In : Inport
  Enable : EnablePort
  Demux : Demux  Outputs=2
  Display : Display
      settings: Format=hex (Stored Integer)
  Display1 : Display
      settings: Format=hex (Stored Integer)
  SPI Master Transfer : c280xlib/SPI Controller Transfer  SPISelect=SPI_A  ClockPolarity=Rising_edge  ClockPhase=No_delay  SPIModule=uint32(0)  Mode=Master  BusSpeed=uint32(1000000)  FirstBitToTransfer=Most significant bit (MSB)  ClockMode=0  BlockFunction=Transfer  EnableRegisterAddress=off  RegisterAddress=0  OutputDataType=int8  OutputDataLength=1  DataBits=16  UseCustomSSPin=Provided by the SPI peripheral  ActiveLowSSPin=Active low  Pin=61
  SPI Master Transfer1 : c280xlib/SPI Controller Transfer  SPISelect=SPI_A  ClockPolarity=Rising_edge  ClockPhase=No_delay  SPIModule=uint32(0)  Mode=Master  BusSpeed=uint32(1000000)  FirstBitToTransfer=Most significant bit (MSB)  ClockMode=0  BlockFunction=Transfer  EnableRegisterAddress=off  RegisterAddress=0  OutputDataType=int8  OutputDataLength=1  DataBits=16  UseCustomSSPin=Provided by the SPI peripheral  ActiveLowSSPin=Active low  Pin=61
  wires:
  Demux/2 -> SPI Master Transfer1/1
  SPI Master Transfer/1 -> Display/1
  SPI Master Transfer1/1 -> Display1/1
  In/1 -> Demux/1
  Demux/1 -> SPI Master Transfer/1

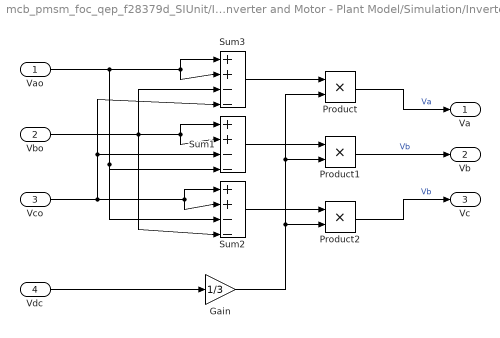
== system mcb_pmsm_foc_qep_f28379d_SIUnit/Inverter and Motor - Plant Model/Simulation/Inverter/Average_Value_Inverter ==
  Vao : Inport
  Vbo : Inport  Port=2
  Vco : Inport  Port=3
  Vdc : Inport  Port=4
  Gain : Gain  Gain=1/3  RndMeth=Simplest  OutDataTypeStr=Inherit: Same as input
  Product : Product  RndMeth=Simplest  OutDataTypeStr=Inherit: Same as first input
  Product1 : Product  RndMeth=Simplest  OutDataTypeStr=Inherit: Same as first input
  Product2 : Product  RndMeth=Simplest  OutDataTypeStr=Inherit: Same as first input
  Sum1 : Sum  Inputs=|++--  RndMeth=Simplest  OutDataTypeStr=Inherit: Same as first input
  Sum2 : Sum  Inputs=|++--  RndMeth=Simplest  OutDataTypeStr=Inherit: Same as first input
  Sum3 : Sum  Inputs=|++--  RndMeth=Simplest  OutDataTypeStr=Inherit: Same as first input
  Va : Outport  VectorParamsAs1DForOutWhenUnconnected=off
  Vb : Outport  Port=2  VectorParamsAs1DForOutWhenUnconnected=off
  Vc : Outport  Port=3  VectorParamsAs1DForOutWhenUnconnected=off
  wires:
  Product1/1 -> Vb/1  "Vb"
  Gain/1 -> Product/2, Product1/2, Product2/2
  Sum2/1 -> Product2/1
  Vao/1 -> Sum3/1, Sum3/2, Sum1/4, Sum2/3
  Product2/1 -> Vc/1  "Vb"
  Sum1/1 -> Product1/1
  Vdc/1 -> Gain/1
  Sum3/1 -> Product/1
  Product/1 -> Va/1  "Va"
  Vco/1 -> Sum3/4, Sum1/3, Sum2/2, Sum2/1
  Vbo/1 -> Sum1/1, Sum1/2, Sum3/3, Sum2/4

== system mcb_pmsm_foc_qep_f28379d_SIUnit/Inverter and Motor - Plant Model/Simulation/Sensor_Measurements/Wrap ==
  in : Inport
  Constant2 : Constant  Value=2*pi  OutDataTypeStr=single  SampleTime=-1
  Mod : Math  Operator=mod
  out : Outport  VectorParamsAs1DForOutWhenUnconnected=off
  wires:
  in/1 -> Mod/1
  Constant2/1 -> Mod/2
  Mod/1 -> out/1

== system mcb_pmsm_foc_qep_f28379d_SIUnit/Serial Receive/Simulation/Data_Conditioning_Tx/Data_Type_Fixed_Point ==
  In1 : Inport
  In2 : Inport  Port=2
  Data Type Conversion : DataTypeConversion  OutDataTypeStr=fixdt(1,32,28)  RndMeth=Simplest  SaturateOnIntegerOverflow=off
  Data Type Conversion1 : DataTypeConversion  OutDataTypeStr=uint32  RndMeth=Simplest  SaturateOnIntegerOverflow=off
  Data Type Conversion3 : DataTypeConversion  OutDataTypeStr=uint32  ConvertRealWorld=Stored Integer (SI)  RndMeth=Simplest  SaturateOnIntegerOverflow=off
  Mux : Mux  Inputs=2
  Data : Outport
  wires:
  In1/1 -> Data Type Conversion/1
  Data Type Conversion3/1 -> Mux/1
  Data Type Conversion/1 -> Data Type Conversion3/1
  In2/1 -> Data Type Conversion1/1
  Data Type Conversion1/1 -> Mux/2
  Mux/1 -> Data/1

== system mcb_pmsm_foc_qep_f28379d_SIUnit/Serial Receive/Simulation/Data_Conditioning_Tx/Data_Type_Float ==
  In1 : Inport
  In2 : Inport  Port=2
  Data Type Conversion2 : DataTypeConversion  OutDataTypeStr=single  RndMeth=Simplest  SaturateOnIntegerOverflow=off
  Mux : Mux  Inputs=2
  Data : Outport
  wires:
  In1/1 -> Mux/1
  Mux/1 -> Data/1
  In2/1 -> Data Type Conversion2/1
  Data Type Conversion2/1 -> Mux/2

== system mcb_pmsm_foc_qep_f28379d_SIUnit/Current Control/Control_System/Closed Loop Control/Current_Controllers/PI_Controller_Id ==
  I_ref : Inport
  I_fb : Inport  Port=2
  Data Store Read1 : DataStoreRead  DataStoreName=Enable  IndexOptions=Index vector (dialog)  Indices=1  OutputSizes=1
  Discrete PI Controller with anti-windup & reset : slpidlib/PID Controller  Controller=PI  Form=Parallel  TimeDomain=Discrete-time  UseExternalTs=off  SampleTime=-1  IntegratorMethod=Forward Euler  FilterMethod=Forward Euler  ControllerParametersSource=external  P=1  I=1  UseKiTs=on  D=0  UseExternalDerivativeSource=off  N=100  UseFilter=on  TunerSelectOption=Transfer Function Based (PID Tuner App)  InitialConditionSource=external  InitialConditionForIntegrator=0  InitialConditionForFilter=0  DifferentiatorICPrevScaledInput=0  ExternalReset=level  TrackingMode=off  Kt=1  LimitOutput=on  SatLimitsSource=internal  UpperSaturationLimit=inverter.V_dc/sqrt(3)  LowerSaturationLimit=-inverter.V_dc/sqrt(3)  LinearizeAsGain=on  AntiWindupMode=clamping  Kb=1  LimitIntegrator=off  UpperIntegratorSaturationLimit=inf  LowerIntegratorSaturationLimit=-inf  RndMeth=Simplest  POutMin=[]  POutMax=[]  IOutMin=[]  IOutMax=[]  DOutMin=[]  DOutMax=[]  NOutMin=[]  NOutMax=[]  SumOutMin=[]  SumOutMax=[]  SaturationOutDataTypeStr=Inherit: Inherit via back propagation  SaturationOutMin=[]  SaturationOutMax=[]  PParamMin=[]  PParamMax=[]  IParamMin=[]  IParamMax=[]  DParamMin=[]  DParamMax=[]  NParamMin=[]  NParamMax=[]  KbParamMin=[]  KbParamMax=[]  KtParamMin=[]  KtParamMax=[]  KbOutMin=[]  KbOutMax=[]  KtOutMin=[]  KtOutMax=[]  IntegratorOutMin=[]  IntegratorOutMax=[]  FilterOutMin=[]  FilterOutMax=[]  SumI1OutMin=[]  SumI1OutMax=[]  SumI2OutMin=[]  SumI2OutMax=[]  SumI3OutMin=[]  SumI3OutMax=[]  SumI4OutMin=[]  SumI4OutMax=[]  SumDOutMin=[]  SumDOutMax=[]  DifferentiatorOutMin=[]  DifferentiatorOutMax=[]  FilterDiffOutCoefMin=[]  FilterDiffOutCoefMax=[]  ReciprocalOutMin=[]  ReciprocalOutMax=[]  SumDenOutMin=[]  SumDenOutMax=[]  SumNumOutMin=[]  SumNumOutMax=[]  DivideOutMin=[]  DivideOutMax=[]  UdiffTsProdOutMin=[]  UdiffTsProdOutMax=[]  NTsProdOutMin=[]  NTsProdOutMax=[]  UintegralTsProdOutMin=[]  UintegralTsProdOutMax=[]  UngainTsProdOutMin=[]  UngainTsProdOutMax=[]  ClampingZeroOutDataTypeStr=Inherit: Inherit via back propagation  ClampingZeroOutMin=[]  ClampingZeroOutMax=[]  FilterDenConstantOutDataTypeStr=Inherit: Inherit via back propagation  FilterDenConstantOutMin=[]  FilterDenConstantOutMax=[]  PCopyOutDataTypeStr=Inherit: Inherit via back propagation  PCopyOutMin=[]  PCopyOutMax=[]  NCopyOutDataTypeStr=Inherit: Inherit via back propagation  NCopyOutMin=[]  NCopyOutMax=[]  IntegratorContinuousStateAttributes=''  IntegratorStateMustResolveToSignalObject=off  IntegratorRTWStateStorageClass=Auto  FilterContinuousStateAttributes=''  FilterStateMustResolveToSignalObject=off  FilterRTWStateStorageClass=Auto  ParallelPVariant=ExternalParameters  IdealPVariant=Disabled  IVariant=ExternalParameters  DVariant=Disabled  IntegratorVariant=Discrete  SatVariant=Enabled  AWVariant=DiscClampingParallel  PCopyVariant=Disabled  TRVariant=Disabled  FdbkBlocksVariant=Forward  IdealPFdbkVariant=Disabled  SatFdbkVariant=Disabled  DerivativeFilterVariant=Disabled  NVariant=Disabled  NCopyVariant=Disabled_SignalSpec  FilterICVariant=Disabled  IntegratorICVariant=ExternalICs  ExternalResetVariant=ExternalReset  TRSumVariant=Passthrough  SumFdbkVariant=Disabled  SumVariant=Sum_PI  TsampFilterVariant=InternalTs  TsampNgainVariant=Passthrough  TsampIntegralVariant=Disabled_SignalSpec  ExternalSaturationOutDataTypeStr=Inherit: Same as second input  DerivativeSourceVariant=Disabled  PreIntVariant=InternalPreInt
      settings: LibrarySourceBlock=mcbcontrolslib/PI Controller
  Ki : Constant  Value=PI_params.Ki_i * Ts  OutDataTypeStr=dataType  SampleTime=-1
  Ki1 : Constant  Value=0  OutDataTypeStr=dataType  SampleTime=-1
  Kp : Constant  Value=PI_params.Kp_i  OutDataTypeStr=dataType  SampleTime=-1
  Logical Operator : Logic  Operator=NOT  IconShape=distinctive  AllPortsSameDT=off  OutDataTypeStr=boolean
  Sum : Sum  Inputs=|+-  OutDataTypeStr=Inherit: Same as first input
  V_ref : Outport  VectorParamsAs1DForOutWhenUnconnected=off
  wires:
  I_ref/1 -> Sum/1
  I_fb/1 -> Sum/2
  Data Store Read1/1 -> Logical Operator/1
  Discrete PI Controller with anti-windup & reset/1 -> V_ref/1
  Sum/1 -> Discrete PI Controller with anti-windup & reset/1
  Kp/1 -> Discrete PI Controller with anti-windup & reset/2
  Ki/1 -> Discrete PI Controller with anti-windup & reset/3
  Logical Operator/1 -> Discrete PI Controller with anti-windup & reset/4
  Ki1/1 -> Discrete PI Controller with anti-windup & reset/5

== system mcb_pmsm_foc_qep_f28379d_SIUnit/Current Control/Control_System/Closed Loop Control/Current_Controllers/PI_Controller_Iq ==
  I_ref : Inport
  I_fb : Inport  Port=2
  Data Store Read1 : DataStoreRead  DataStoreName=Enable  IndexOptions=Index vector (dialog)  Indices=1  OutputSizes=1
  Discrete PI Controller with anti-windup & reset : slpidlib/PID Controller  Controller=PI  Form=Parallel  TimeDomain=Discrete-time  UseExternalTs=off  SampleTime=-1  IntegratorMethod=Forward Euler  FilterMethod=Forward Euler  ControllerParametersSource=external  P=1  I=1  UseKiTs=on  D=0  UseExternalDerivativeSource=off  N=100  UseFilter=on  TunerSelectOption=Transfer Function Based (PID Tuner App)  InitialConditionSource=external  InitialConditionForIntegrator=0  InitialConditionForFilter=0  DifferentiatorICPrevScaledInput=0  ExternalReset=level  TrackingMode=off  Kt=1  LimitOutput=on  SatLimitsSource=internal  UpperSaturationLimit=inverter.V_dc/sqrt(3)  LowerSaturationLimit=-inverter.V_dc/sqrt(3)  LinearizeAsGain=on  AntiWindupMode=clamping  Kb=1  LimitIntegrator=off  UpperIntegratorSaturationLimit=inf  LowerIntegratorSaturationLimit=-inf  RndMeth=Simplest  POutMin=[]  POutMax=[]  IOutMin=[]  IOutMax=[]  DOutMin=[]  DOutMax=[]  NOutMin=[]  NOutMax=[]  SumOutMin=[]  SumOutMax=[]  SaturationOutDataTypeStr=Inherit: Inherit via back propagation  SaturationOutMin=[]  SaturationOutMax=[]  PParamMin=[]  PParamMax=[]  IParamMin=[]  IParamMax=[]  DParamMin=[]  DParamMax=[]  NParamMin=[]  NParamMax=[]  KbParamMin=[]  KbParamMax=[]  KtParamMin=[]  KtParamMax=[]  KbOutMin=[]  KbOutMax=[]  KtOutMin=[]  KtOutMax=[]  IntegratorOutMin=[]  IntegratorOutMax=[]  FilterOutMin=[]  FilterOutMax=[]  SumI1OutMin=[]  SumI1OutMax=[]  SumI2OutMin=[]  SumI2OutMax=[]  SumI3OutMin=[]  SumI3OutMax=[]  SumI4OutMin=[]  SumI4OutMax=[]  SumDOutMin=[]  SumDOutMax=[]  DifferentiatorOutMin=[]  DifferentiatorOutMax=[]  FilterDiffOutCoefMin=[]  FilterDiffOutCoefMax=[]  ReciprocalOutMin=[]  ReciprocalOutMax=[]  SumDenOutMin=[]  SumDenOutMax=[]  SumNumOutMin=[]  SumNumOutMax=[]  DivideOutMin=[]  DivideOutMax=[]  UdiffTsProdOutMin=[]  UdiffTsProdOutMax=[]  NTsProdOutMin=[]  NTsProdOutMax=[]  UintegralTsProdOutMin=[]  UintegralTsProdOutMax=[]  UngainTsProdOutMin=[]  UngainTsProdOutMax=[]  ClampingZeroOutDataTypeStr=Inherit: Inherit via back propagation  ClampingZeroOutMin=[]  ClampingZeroOutMax=[]  FilterDenConstantOutDataTypeStr=Inherit: Inherit via back propagation  FilterDenConstantOutMin=[]  FilterDenConstantOutMax=[]  PCopyOutDataTypeStr=Inherit: Inherit via back propagation  PCopyOutMin=[]  PCopyOutMax=[]  NCopyOutDataTypeStr=Inherit: Inherit via back propagation  NCopyOutMin=[]  NCopyOutMax=[]  IntegratorContinuousStateAttributes=''  IntegratorStateMustResolveToSignalObject=off  IntegratorRTWStateStorageClass=Auto  FilterContinuousStateAttributes=''  FilterStateMustResolveToSignalObject=off  FilterRTWStateStorageClass=Auto  ParallelPVariant=ExternalParameters  IdealPVariant=Disabled  IVariant=ExternalParameters  DVariant=Disabled  IntegratorVariant=Discrete  SatVariant=Enabled  AWVariant=DiscClampingParallel  PCopyVariant=Disabled  TRVariant=Disabled  FdbkBlocksVariant=Forward  IdealPFdbkVariant=Disabled  SatFdbkVariant=Disabled  DerivativeFilterVariant=Disabled  NVariant=Disabled  NCopyVariant=Disabled_SignalSpec  FilterICVariant=Disabled  IntegratorICVariant=ExternalICs  ExternalResetVariant=ExternalReset  TRSumVariant=Passthrough  SumFdbkVariant=Disabled  SumVariant=Sum_PI  TsampFilterVariant=InternalTs  TsampNgainVariant=Passthrough  TsampIntegralVariant=Disabled_SignalSpec  ExternalSaturationOutDataTypeStr=Inherit: Same as second input  DerivativeSourceVariant=Disabled  PreIntVariant=InternalPreInt
      settings: LibrarySourceBlock=mcbcontrolslib/PI Controller
  Ki : Constant  Value=PI_params.Ki_i * Ts  OutDataTypeStr=dataType  SampleTime=-1
  Kp : Constant  Value=PI_params.Kp_i  OutDataTypeStr=dataType  SampleTime=-1
  Kp1 : Constant  Value=0  OutDataTypeStr=dataType  SampleTime=-1
  Logical Operator : Logic  Operator=NOT  IconShape=distinctive  AllPortsSameDT=off  OutDataTypeStr=boolean
  Sum : Sum  Inputs=|+-  OutDataTypeStr=Inherit: Same as first input
  V_ref : Outport  VectorParamsAs1DForOutWhenUnconnected=off
  wires:
  Discrete PI Controller with anti-windup & reset/1 -> V_ref/1
  Data Store Read1/1 -> Logical Operator/1
  I_fb/1 -> Sum/2
  I_ref/1 -> Sum/1
  Kp/1 -> Discrete PI Controller with anti-windup & reset/2
  Sum/1 -> Discrete PI Controller with anti-windup & reset/1
  Ki/1 -> Discrete PI Controller with anti-windup & reset/3
  Logical Operator/1 -> Discrete PI Controller with anti-windup & reset/4
  Kp1/1 -> Discrete PI Controller with anti-windup & reset/5

== system mcb_pmsm_foc_qep_f28379d_SIUnit/Hardware Init/Code Generation/Calculate ADC Offset /For Iterator Subsystem/If Action Subsystem ==
  In1 : Inport
  In2 : Inport  Port=2
  Action Port : ActionPort  ActionPortLabel=if(u1 > 8)
  Memory : Memory  InheritSampleTime=on
  Memory1 : Memory  InheritSampleTime=on
  Sum : Sum
  Sum1 : Sum
  Out1 : Outport
  Out2 : Outport  Port=2
  wires:
  In1/1 -> Sum/1
  Sum/1 -> Out1/1, Memory/1
  In2/1 -> Sum1/1
  Memory/1 -> Sum/2
  Sum1/1 -> Out2/1, Memory1/1
  Memory1/1 -> Sum1/2
